simulink model "passband_72_channels_1Updated"  (R2026a)
settings: Solver=FixedStepDiscrete  StopTime=0.3  FixedStep=1e-7
libraries: commdigbbndpm3 x2, slctrl_signal x2, simulink x1, commsink2 x1, dspsigops x1, commrandsrc3 x1
settings Model: Creator=MADHAV  LastModifiedBy=Kian

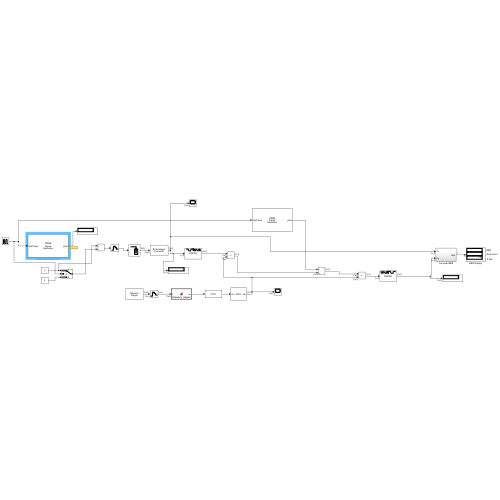
[thumbnail: Simulink's stored preview of the top-level diagram]
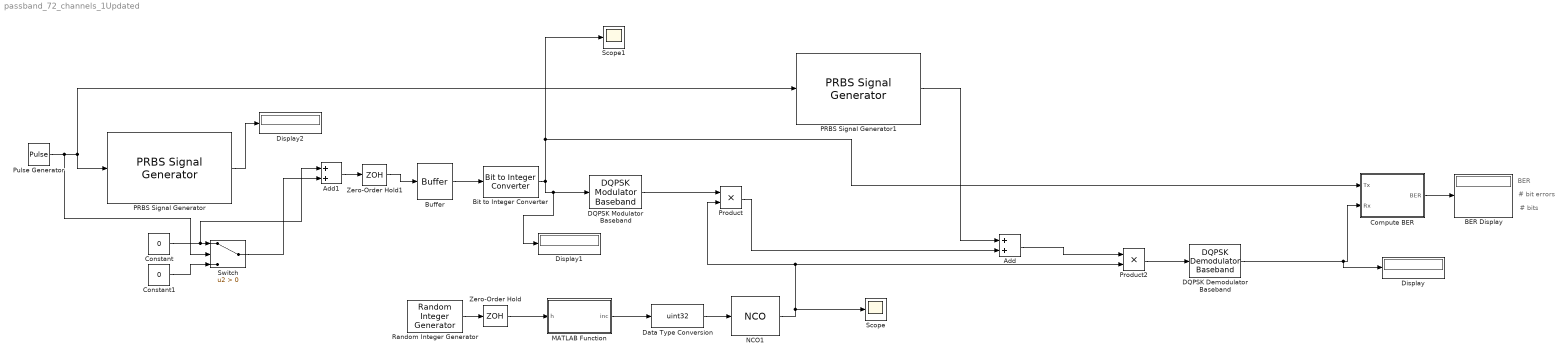
== system passband_72_channels_1Updated ==
  note: # bits
  note: BER
  note: # bit errors
  Add : Sum
  Add1 : Sum
  BER Display : Display
  Bit to Integer Converter : simulink/Logic and Bit Operations/Bit to Integer Converter  nbits=2  bitOrder=MSB first  signedOutputValues=Unsigned  outDtype=Inherit via internal rule  outDtypeSigned=Inherit via internal rule
  Buffer : Buffer  N=2  OutputFrames=off
  Compute BER : Subsystem
  Constant : Constant  Value=0
  Constant1 : Constant  Value=0
  DQPSK Demodulator Baseband : commdigbbndpm3/DQPSK Demodulator Baseband  OutType=Integer  Dec=Gray  Ph=pi/4  outDtype1=Inherit via internal rule  outDtype2=Inherit via internal rule
  DQPSK Modulator Baseband : commdigbbndpm3/DQPSK Modulator Baseband  InType=Integer  Enc=Gray  Ph=pi/4  outDtype=double
  Data Type Conversion : DataTypeConversion  OutDataTypeStr=uint32  SaturateOnIntegerOverflow=off  RndMeth=Floor
  Display : Display
  Display1 : Display
  Display2 : Display
  MATLAB Function : MATLAB Function  TreatAsAtomicUnit=on
  NCO1 : dspsigops/NCO  AccIncSrc=Input port  AccInc=100  PhaseOffsetSrc=Specify via dialog  PhaseOffset=0  AccumWL=16  HasDither=on  DitherWL=4  PNgeneratorLength=19  HasPhaseQuantizer=on  TableDepth=12  HasOutputPhaseError=off  Formula=Sine  DataType=Binary point scaling  OutputWL=16  OutputFL=14  CompMethod=Table lookup (no interpolation)  SampleTime=1  SamplesPerFrame=1  OutputFrames=off
  PRBS Signal Generator : slctrl_signal/PRBS Signal Generator  DiscreteTs=5e-7  BlockDataType=double  SignalSource=Block parameters  Frequencies=[9.784e-11 2.5e-7]  FreqUnits=Hz  Amplitudes=1  NumOfFreq=3  NumOfPRBSPeriod=10  UseAutogenNumOfPRBSPeriod=off  PRBSSignalOrder=9  UseAutogenPRBSSignalOrder=off  UseExternalTs=off  CompiledTsChoice=InternalTs
  PRBS Signal Generator1 : slctrl_signal/PRBS Signal Generator  DiscreteTs=5e-7  BlockDataType=double  SignalSource=Block parameters  Frequencies=[2*pi*1000 2*pi*900e3]  FreqUnits=rad/s  Amplitudes=1  NumOfFreq=3  NumOfPRBSPeriod=10  UseAutogenNumOfPRBSPeriod=off  PRBSSignalOrder=15  UseAutogenPRBSSignalOrder=off  UseExternalTs=off  CompiledTsChoice=InternalTs
  Product : Product  RndMeth=Zero
  Product2 : Product
  Pulse Generator : DiscretePulseGenerator  PulseType=Time based  Period=1  PulseWidth=5e-5
  Random Integer Generator : commrandsrc3/Random Integer Generator  SetSize=71  SeedSource=Auto  Seed=12345  SampleTime=1e-3  SamplesPerFrame=1  OutputDataType=double  SimulateUsing=Interpreted execution
  Scope : Scope
  Scope1 : Scope
      settings: ActiveDisplayYMinimum=-0.2401601169685296  ActiveDisplayYMaximum=0.25443494131113592
  Switch : Switch  Criteria=u2 > Threshold  SaturateOnIntegerOverflow=off  InputSameDT=off
  Zero-Order Hold : ZeroOrderHold  SampleTime=5e-6
  Zero-Order Hold1 : ZeroOrderHold  SampleTime=5e-7
  wires:
  Zero-Order Hold/1 -> MATLAB Function/1(h)
  Data Type Conversion/1 -> NCO1/1
  Random Integer Generator/1 -> Zero-Order Hold/1
  MATLAB Function/1(inc) -> Data Type Conversion/1
  DQPSK Modulator Baseband/1 -> Product/1
  Product2/1 -> DQPSK Demodulator Baseband/1
  Add/1 -> Product2/1
  Compute BER/1(BER) -> BER Display/1
  NCO1/1 -> Product/2, Product2/2, Scope/1
  Product/1 -> Add/2
  PRBS Signal Generator1/1 -> Add/1
  Pulse Generator/1 -> Switch/2, PRBS Signal Generator1/1, PRBS Signal Generator/1
  DQPSK Demodulator Baseband/1 -> Display/1, Compute BER/2(Rx)
  Bit to Integer Converter/1 -> Display1/1, DQPSK Modulator Baseband/1, Compute BER/1(Tx), Scope1/1
  Buffer/1 -> Bit to Integer Converter/1
  Zero-Order Hold1/1 -> Buffer/1
  Add1/1 -> Zero-Order Hold1/1
  Constant/1 -> Add1/1, Switch/1
  Switch/1 -> Add1/2
  Constant1/1 -> Switch/3
  PRBS Signal Generator/1 -> Display2/1

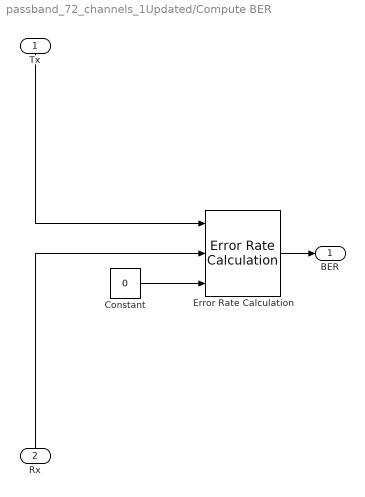
== system passband_72_channels_1Updated/Compute BER ==
  Tx : Inport
  Rx : Inport  Port=2
  Constant : Constant  Value=0  SampleTime=1e-4
  Error Rate Calculation : commsink2/Error Rate Calculation  N=16  st_delay=0  cp_mode=Entire frame  subframe=[]  PMode=Port  WsName=ErrorVec  RsMode2=on  stop=off  numErr=100  maxBits=1e6
  BER : Outport  VectorParamsAs1DForOutWhenUnconnected=off
  wires:
  Error Rate Calculation/1 -> BER/1
  Constant/1 -> Error Rate Calculation/3
  Tx/1 -> Error Rate Calculation/1
  Rx/1 -> Error Rate Calculation/2

== matlab function passband_72_channels_1Updated/MATLAB Function ==
  data: h input; inc output
function inc = frequency_mapper(h)

% Convert hop index (0 to 71) to frequency
f = 1000 + h*1000;

% Convert frequency to NCO phase increment
inc = floor(f*65536/200000);
